simulink model "quadcopter_ctrl_wrench"  (R2024b)
settings: Solver=VariableStepAuto  StartTime=0.0  StopTime=60  RelTol=1e-3
values from neighbouring files (symbols this model uses):
  Ts = 0.001    [params.m]    (also in traj_gen.m)
libraries: robotcorelib x1, uavutilslib x1
settings Model: Creator=feder  LastModifiedBy=mattr

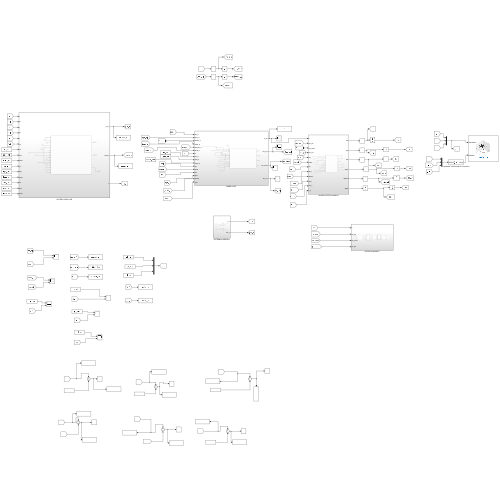
[thumbnail: Simulink's stored preview of the top-level diagram]
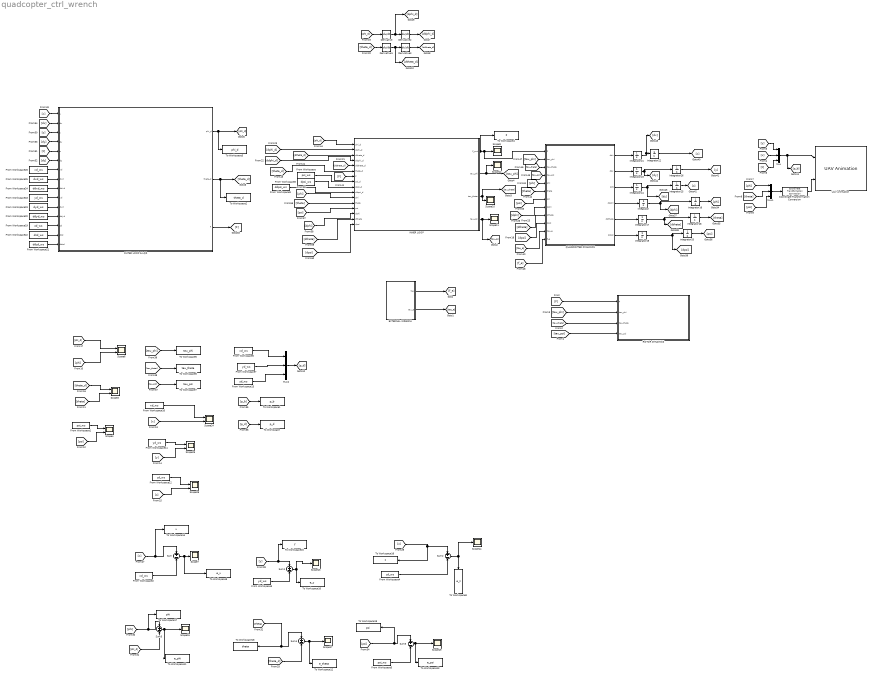
== system quadcopter_ctrl_wrench ==
  Coordinate Transformation Conversion : robotcorelib/Coordinate Transformation Conversion  InputRepresentation=Euler Angles  InputEulerSequence=XYZ  ShowTrVecInputPort=on  OutputRepresentation=Quaternion  OutputEulerSequence=ZYX  ShowTrVecOutputPort=on  SimulateUsing=Interpreted execution
  Derivative : Derivative
  Derivative1 : Derivative  CoefficientInTFapproximation=Ts
  Derivative2 : Derivative
  Derivative3 : Derivative  CoefficientInTFapproximation=Ts
  EXTERNAL WRENCH : Subsystem
  From Workspace : FromWorkspace  VariableName=psi_ws
  From Workspace1 : FromWorkspace  VariableName=psi_ws
  From Workspace{2,6,10,26} (4 alike) : FromWorkspace  VariableName=xd_ws
  From Workspace{3,7,11,18} (4 alike) : FromWorkspace  VariableName=yd_ws
  From Workspace{4,12..13,19} (4 alike) : FromWorkspace  VariableName=zd_ws
  From Workspace20 : FromWorkspace  VariableName=ddyd_ws
  From Workspace21 : FromWorkspace  VariableName=ddzd_ws
  From Workspace22 : FromWorkspace  VariableName=dzd_ws
  From Workspace23 : FromWorkspace  VariableName=dyd_ws
  From Workspace24 : FromWorkspace  VariableName=ddxd_ws
  From Workspace25 : FromWorkspace  VariableName=dxd_ws
  From Workspace5 : FromWorkspace  VariableName=psi_ws
  From Workspace8 : FromWorkspace  VariableName=dpsi_ws
  From Workspace9 : FromWorkspace  VariableName=ddpsi_ws
  INNER LOOP : Subsystem
  Integrator{,17,19,21..26} (9 alike) : Integrator
  Integrator16 : Integrator  InitialCondition=0.09
  Integrator18 : Integrator  InitialCondition=-0.0100316
  Integrator20 : Integrator  InitialCondition=pi/4
  Mux : Mux  Inputs=3
  Mux1 : Mux  Inputs=3
  Mux2 : Mux  Inputs=3
  OUTER LOOP & LQR : Subsystem
  QUADCOPTER DYNAMICS : Subsystem
  ROTOR DYNAMICS : Subsystem
  Scope{7,9..15,17,19} (10 alike) : Scope
  Scope{3..4,6,24..26} (6 alike) : Scope  NumInputPorts=2
  Sum{,1..5} (6 alike) : Sum  Inputs=+-
  To Workspace : ToWorkspace  VariableName=p_d  SaveFormat=Timeseries  SampleTime=-1
  To Workspace1 : ToWorkspace  VariableName=p_b  SaveFormat=Timeseries  SampleTime=-1
  To Workspace10 : ToWorkspace  VariableName=e_y  SaveFormat=Timeseries  SampleTime=-1
  To Workspace11 : ToWorkspace  VariableName=e_phi  SaveFormat=Timeseries  SampleTime=-1
  To Workspace12 : ToWorkspace  VariableName=e_theta  SaveFormat=Timeseries  SampleTime=-1
  To Workspace13 : ToWorkspace  VariableName=e_psi  SaveFormat=Timeseries  SampleTime=-1
  To Workspace14 : ToWorkspace  VariableName=x  SaveFormat=Timeseries  SampleTime=-1
  To Workspace15 : ToWorkspace  VariableName=y  SaveFormat=Timeseries  SampleTime=-1
  To Workspace16 : ToWorkspace  VariableName=z  SaveFormat=Timeseries  SampleTime=-1
  To Workspace17 : ToWorkspace  VariableName=phi  SaveFormat=Timeseries  SampleTime=-1
  To Workspace18 : ToWorkspace  VariableName=theta  SaveFormat=Timeseries  SampleTime=-1
  To Workspace19 : ToWorkspace  VariableName=psi  SaveFormat=Timeseries  SampleTime=-1
  To Workspace2 : ToWorkspace  VariableName=theta_d  SaveFormat=Timeseries  SampleTime=-1
  To Workspace3 : ToWorkspace  VariableName=phi_d  SaveFormat=Timeseries  SampleTime=-1
  To Workspace4 : ToWorkspace  VariableName=F  SaveFormat=Timeseries  SampleTime=-1
  To Workspace5 : ToWorkspace  VariableName=tau_phi  SaveFormat=Timeseries  SampleTime=-1
  To Workspace6 : ToWorkspace  VariableName=tau_theta  SaveFormat=Timeseries  SampleTime=-1
  To Workspace7 : ToWorkspace  VariableName=tau_psi  SaveFormat=Timeseries  SampleTime=-1
  To Workspace8 : ToWorkspace  VariableName=e_z  SaveFormat=Timeseries  SampleTime=-1
  To Workspace9 : ToWorkspace  VariableName=e_x  SaveFormat=Timeseries  SampleTime=-1
  UAV Animation : uavutilslib/UAV Animation  NumUAV=1  DynamicUAVConfig=off  UAVType=Multirotor  UAVSize=1  UAVColor=[1 0 0]  UAVTrajectoryAlpha=1  InertialZDirection=Up  RotationFormat=Quaternion  DrawMarkers=off  SampleTime=0.01
  wires:
  [z] -> Sum2/1, To Workspace16/1
  From Workspace4/1 -> Sum2/2
  Sum2/1 -> Scope14/1, To Workspace8/1
  [x] -> Scope24/2
  From Workspace11/1 -> Scope25/1
  From Workspace10/1 -> Scope24/1
  [phi_d] -> INNER LOOP/1(phi_d)
  [tau_theta] -> QUADCOPTER DYNAMICS/3(tau_theta)
  [theta] -> Scope3/2
  [theta_d] -> Scope3/1
  Mux2/1 -> [p_d]
  [ddtheta_d] -> INNER LOOP/5(ddtheta_d)
  OUTER LOOP & LQR/3(F) -> [F]
  From Workspace21/1 -> OUTER LOOP & LQR/15(ddzd)
  From Workspace19/1 -> OUTER LOOP & LQR/13(zd)
  From Workspace18/1 -> OUTER LOOP & LQR/10(yd)
  [z] -> OUTER LOOP & LQR/5(z)
  From Workspace20/1 -> OUTER LOOP & LQR/12(ddyd)
  [y] -> OUTER LOOP & LQR/3(y)
  [dx] -> OUTER LOOP & LQR/2(dx)
  [x] -> OUTER LOOP & LQR/1(x)
  [tau_psi] -> QUADCOPTER DYNAMICS/4(tau_psi)
  Sum/1 -> To Workspace9/1, Scope7/1
  [z] -> Scope26/2
  [x] -> To Workspace14/1, Sum/1
  [y] -> To Workspace15/1, Sum1/1
  From Workspace3/1 -> Sum1/2
  [phi_d] -> Sum3/2
  Sum1/1 -> Scope13/1, To Workspace10/1
  Sum3/1 -> To Workspace11/1, Scope15/1
  From Workspace2/1 -> Sum/2
  [psi] -> Mux1/3
  QUADCOPTER DYNAMICS/1(ddx) -> Integrator21/1
  QUADCOPTER DYNAMICS/5(ddtheta) -> Integrator17/1
  QUADCOPTER DYNAMICS/4(ddphi) -> Integrator/1
  [dpsi] -> QUADCOPTER DYNAMICS/10(dpsi)
  QUADCOPTER DYNAMICS/3(ddz) -> Integrator24/1
  [y] -> Scope25/2
  QUADCOPTER DYNAMICS/6(ddpsi) -> Integrator19/1
  QUADCOPTER DYNAMICS/2(ddy) -> Integrator23/1
  [theta] -> QUADCOPTER DYNAMICS/6(theta)
  [phi] -> QUADCOPTER DYNAMICS/5(phi)
  [dtheta] -> QUADCOPTER DYNAMICS/9(dtheta)
  [dphi] -> QUADCOPTER DYNAMICS/8(dphi)
  [psi] -> QUADCOPTER DYNAMICS/7(psi)
  [dpsi] -> INNER LOOP/16(dpsi)
  INNER LOOP/3(tau_theta) -> Scope10/1, [tau_theta]
  INNER LOOP/2(tau_phi) -> [tau_phi], Scope12/1
  INNER LOOP/4(tau_psi) -> Scope11/1, [tau_psi]
  INNER LOOP/1(F_out) -> To Workspace4/1, QUADCOPTER DYNAMICS/1(F), Scope9/1
  [theta] -> INNER LOOP/12(theta)
  [psi] -> INNER LOOP/13(psi)
  [dtheta] -> INNER LOOP/15(dtheta)
  [phi] -> INNER LOOP/11(phi)
  From Workspace9/1 -> INNER LOOP/10(ddpsi_d)
  From Workspace8/1 -> INNER LOOP/9(dpsi_d)
  From Workspace/1 -> INNER LOOP/8(psi_d)
  [F] -> INNER LOOP/7(F)
  [ddphi_d] -> INNER LOOP/4(ddphi_d)
  [dtheta_d] -> INNER LOOP/3(dtheta_d)
  [tau_phi] -> QUADCOPTER DYNAMICS/2(tau_phi)
  [dz] -> OUTER LOOP & LQR/6(dz)
  From Workspace1/1 -> Scope4/1
  [theta_d] -> Derivative1/1
  [phi] -> Scope6/2
  [y] -> Mux/1
  [phi] -> Mux1/1
  Integrator20/1 -> [psi]
  Derivative/1 -> [dphi_d], Derivative2/1
  Integrator25/1 -> [z]
  Mux1/1 -> Coordinate Transformation Conversion/1
  Integrator19/1 -> [dpsi], Integrator20/1
  From Workspace24/1 -> OUTER LOOP & LQR/9(ddxd)
  [dphi_d] -> INNER LOOP/2(dphi_d)
  Integrator26/1 -> [y]
  Integrator/1 -> [dphi], Integrator16/1
  [phi_d] -> Derivative/1
  Integrator17/1 -> [dtheta], Integrator18/1
  [theta] -> Mux1/2
  Integrator18/1 -> [theta]
  From Workspace22/1 -> OUTER LOOP & LQR/14(dzd)
  From Workspace25/1 -> OUTER LOOP & LQR/8(dxd)
  Integrator21/1 -> [dx], Integrator22/1
  From Workspace23/1 -> OUTER LOOP & LQR/11(dyd)
  Integrator16/1 -> [phi]
  Derivative2/1 -> [ddphi_d]
  Coordinate Transformation Conversion/1 -> UAV Animation/2
  Derivative3/1 -> [ddtheta_d]
  [dy] -> OUTER LOOP & LQR/4(dy)
  [phi] -> To Workspace17/1, Sum3/1
  From Workspace12/1 -> Scope26/1
  [tau_phi] -> To Workspace5/1
  Derivative1/1 -> [dtheta_d], Derivative3/1
  Integrator22/1 -> [x]
  [z] -> Mux/3
  [x] -> Mux/2
  Integrator23/1 -> [dy], Integrator26/1
  [theta] -> To Workspace18/1, Sum4/1
  [theta_d] -> Sum4/2
  Mux/1 -> [p_b], UAV Animation/1
  From Workspace5/1 -> Sum5/2
  Integrator24/1 -> [dz], Integrator25/1
  [dphi] -> INNER LOOP/14(dphi)
  Sum4/1 -> To Workspace12/1, Scope17/1
  [psi] -> Sum5/1, To Workspace19/1
  From Workspace7/1 -> Mux2/2
  [p_d] -> To Workspace/1
  OUTER LOOP & LQR/2(theta_d) -> To Workspace2/1, [theta_d]
  [tau_theta] -> To Workspace6/1
  From Workspace26/1 -> OUTER LOOP & LQR/7(xd)
  [p_b] -> To Workspace1/1
  From Workspace13/1 -> Mux2/3
  [F] -> ROTOR DYNAMICS/1(F)
  [tau_theta] -> ROTOR DYNAMICS/3(tau_theta)
  [tau_psi] -> ROTOR DYNAMICS/4(tau_psi)
  [phi_d] -> Scope6/1
  Sum5/1 -> To Workspace13/1, Scope19/1
  [tau_phi] -> ROTOR DYNAMICS/2(tau_phi)
  [tau_psi] -> To Workspace7/1
  OUTER LOOP & LQR/1(phi_d) -> [phi_d], To Workspace3/1
  [psi] -> Scope4/2
  From Workspace6/1 -> Mux2/1
  [theta_d] -> INNER LOOP/6(theta_d)
  [tau_e] -> QUADCOPTER DYNAMICS/11(tau_e)
  [f_e] -> QUADCOPTER DYNAMICS/12(f_e)
  EXTERNAL WRENCH/1(f_e) -> [f_e]
  EXTERNAL WRENCH/2(tau_e) -> [tau_e]

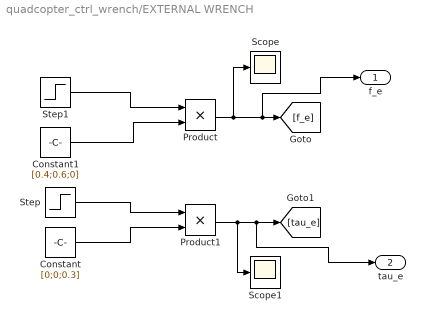
== system quadcopter_ctrl_wrench/EXTERNAL WRENCH ==
  Constant : Constant  Value=[0;0;0.3]  SampleTime=Ts
  Constant1 : Constant  Value=[0.4;0.6;0]  SampleTime=Ts
  Product : Product
  Product1 : Product
  Scope : Scope
  Scope1 : Scope
  Step : Step  Time=12  SampleTime=Ts
  Step1 : Step  Time=12  SampleTime=Ts
  f_e : Outport
  tau_e : Outport  Port=2
  wires:
  Product/1 -> Scope/1, f_e/1, [f_e]
  Product1/1 -> Scope1/1, tau_e/1, [tau_e]
  Step1/1 -> Product/1
  Constant1/1 -> Product/2
  Step/1 -> Product1/1
  Constant/1 -> Product1/2

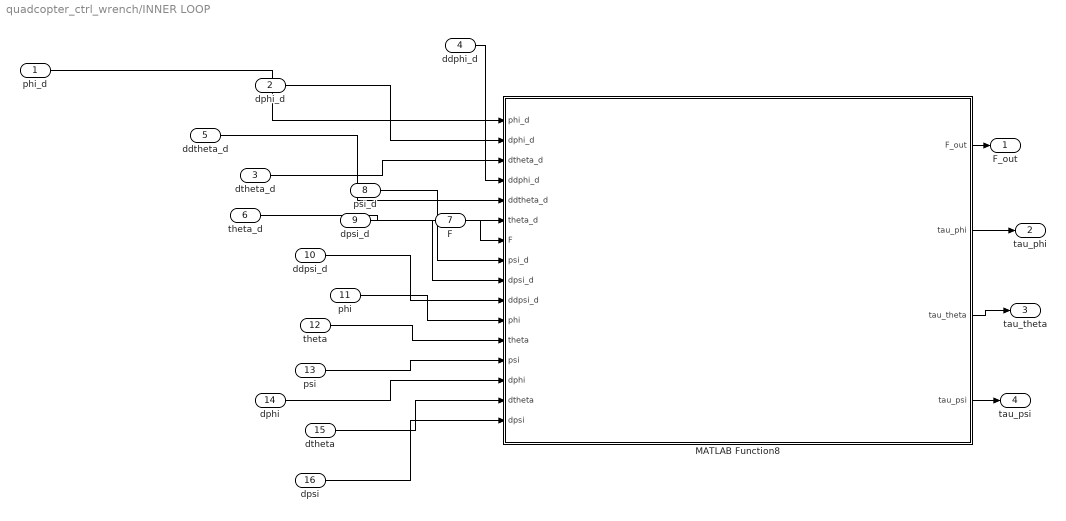
== system quadcopter_ctrl_wrench/INNER LOOP ==
  phi_d : Inport
  dphi_d : Inport  Port=2
  dtheta_d : Inport  Port=3
  ddphi_d : Inport  Port=4
  ddtheta_d : Inport  Port=5
  theta_d : Inport  Port=6
  F : Inport  Port=7
  psi_d : Inport  Port=8
  dpsi_d : Inport  Port=9
  ddpsi_d : Inport  Port=10
  phi : Inport  Port=11
  theta : Inport  Port=12
  psi : Inport  Port=13
  dphi : Inport  Port=14
  dtheta : Inport  Port=15
  dpsi : Inport  Port=16
  MATLAB Function8 : MATLAB Function  TreatAsAtomicUnit=on
  F_out : Outport
  tau_phi : Outport  Port=2
  tau_theta : Outport  Port=3
  tau_psi : Outport  Port=4
  wires:
  ddphi_d/1 -> MATLAB Function8/4(ddphi_d)
  psi_d/1 -> MATLAB Function8/8(psi_d)
  ddpsi_d/1 -> MATLAB Function8/10(ddpsi_d)
  F/1 -> MATLAB Function8/7(F)
  psi/1 -> MATLAB Function8/13(psi)
  dphi_d/1 -> MATLAB Function8/2(dphi_d)
  dphi/1 -> MATLAB Function8/14(dphi)
  phi_d/1 -> MATLAB Function8/1(phi_d)
  MATLAB Function8/1(F_out) -> F_out/1
  phi/1 -> MATLAB Function8/11(phi)
  dpsi_d/1 -> MATLAB Function8/9(dpsi_d)
  ddtheta_d/1 -> MATLAB Function8/5(ddtheta_d)
  theta/1 -> MATLAB Function8/12(theta)
  MATLAB Function8/2(tau_phi) -> tau_phi/1
  MATLAB Function8/3(tau_theta) -> tau_theta/1
  dtheta_d/1 -> MATLAB Function8/3(dtheta_d)
  dtheta/1 -> MATLAB Function8/15(dtheta)
  MATLAB Function8/4(tau_psi) -> tau_psi/1
  theta_d/1 -> MATLAB Function8/6(theta_d)
  dpsi/1 -> MATLAB Function8/16(dpsi)

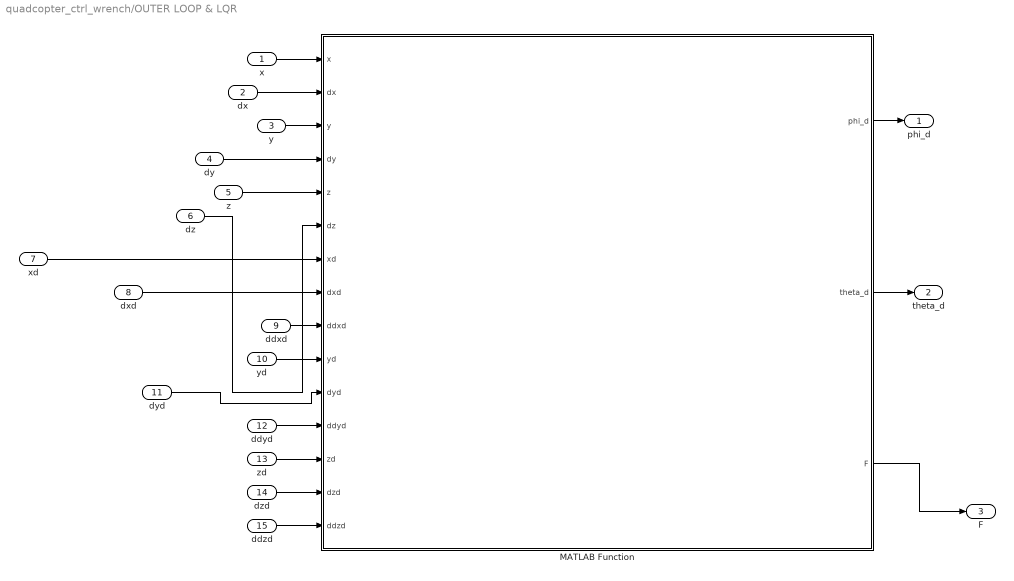
== system quadcopter_ctrl_wrench/OUTER LOOP & LQR ==
  x : Inport
  dx : Inport  Port=2
  y : Inport  Port=3
  dy : Inport  Port=4
  z : Inport  Port=5
  dz : Inport  Port=6
  xd : Inport  Port=7
  dxd : Inport  Port=8
  ddxd : Inport  Port=9
  yd : Inport  Port=10
  dyd : Inport  Port=11
  ddyd : Inport  Port=12
  zd : Inport  Port=13
  dzd : Inport  Port=14
  ddzd : Inport  Port=15
  MATLAB Function : MATLAB Function  TreatAsAtomicUnit=on
  phi_d : Outport
  theta_d : Outport  Port=2
  F : Outport  Port=3
  wires:
  zd/1 -> MATLAB Function/13(zd)
  MATLAB Function/1(phi_d) -> phi_d/1
  xd/1 -> MATLAB Function/7(xd)
  dxd/1 -> MATLAB Function/8(dxd)
  dy/1 -> MATLAB Function/4(dy)
  MATLAB Function/2(theta_d) -> theta_d/1
  dyd/1 -> MATLAB Function/11(dyd)
  ddzd/1 -> MATLAB Function/15(ddzd)
  dz/1 -> MATLAB Function/6(dz)
  yd/1 -> MATLAB Function/10(yd)
  dx/1 -> MATLAB Function/2(dx)
  dzd/1 -> MATLAB Function/14(dzd)
  y/1 -> MATLAB Function/3(y)
  ddxd/1 -> MATLAB Function/9(ddxd)
  z/1 -> MATLAB Function/5(z)
  ddyd/1 -> MATLAB Function/12(ddyd)
  x/1 -> MATLAB Function/1(x)
  MATLAB Function/3(F) -> F/1

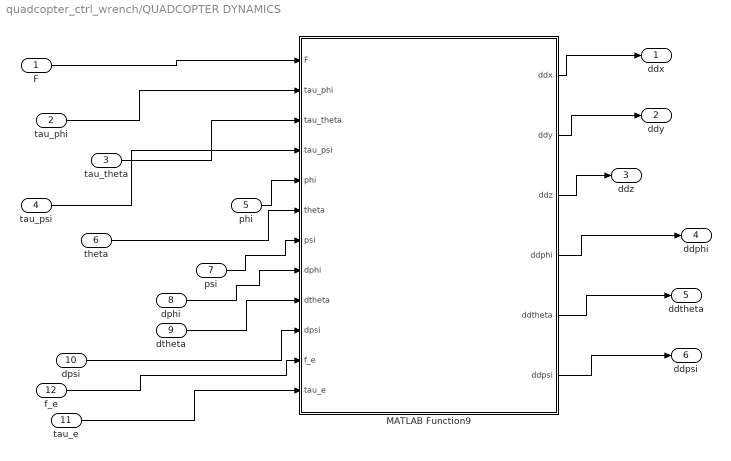
== system quadcopter_ctrl_wrench/QUADCOPTER DYNAMICS ==
  F : Inport
  tau_phi : Inport  Port=2
  tau_theta : Inport  Port=3
  tau_psi : Inport  Port=4
  phi : Inport  Port=5
  theta : Inport  Port=6
  psi : Inport  Port=7
  dphi : Inport  Port=8
  dtheta : Inport  Port=9
  dpsi : Inport  Port=10
  tau_e : Inport  Port=11
  f_e : Inport  Port=12
  MATLAB Function9 : MATLAB Function  TreatAsAtomicUnit=on
  ddx : Outport
  ddy : Outport  Port=2
  ddz : Outport  Port=3
  ddphi : Outport  Port=4
  ddtheta : Outport  Port=5
  ddpsi : Outport  Port=6
  wires:
  dphi/1 -> MATLAB Function9/8(dphi)
  MATLAB Function9/6(ddpsi) -> ddpsi/1
  phi/1 -> MATLAB Function9/5(phi)
  MATLAB Function9/2(ddy) -> ddy/1
  tau_phi/1 -> MATLAB Function9/2(tau_phi)
  MATLAB Function9/4(ddphi) -> ddphi/1
  F/1 -> MATLAB Function9/1(F)
  dtheta/1 -> MATLAB Function9/9(dtheta)
  MATLAB Function9/3(ddz) -> ddz/1
  tau_theta/1 -> MATLAB Function9/3(tau_theta)
  MATLAB Function9/1(ddx) -> ddx/1
  MATLAB Function9/5(ddtheta) -> ddtheta/1
  theta/1 -> MATLAB Function9/6(theta)
  dpsi/1 -> MATLAB Function9/10(dpsi)
  tau_psi/1 -> MATLAB Function9/4(tau_psi)
  psi/1 -> MATLAB Function9/7(psi)
  tau_e/1 -> MATLAB Function9/12(tau_e)
  f_e/1 -> MATLAB Function9/11(f_e)

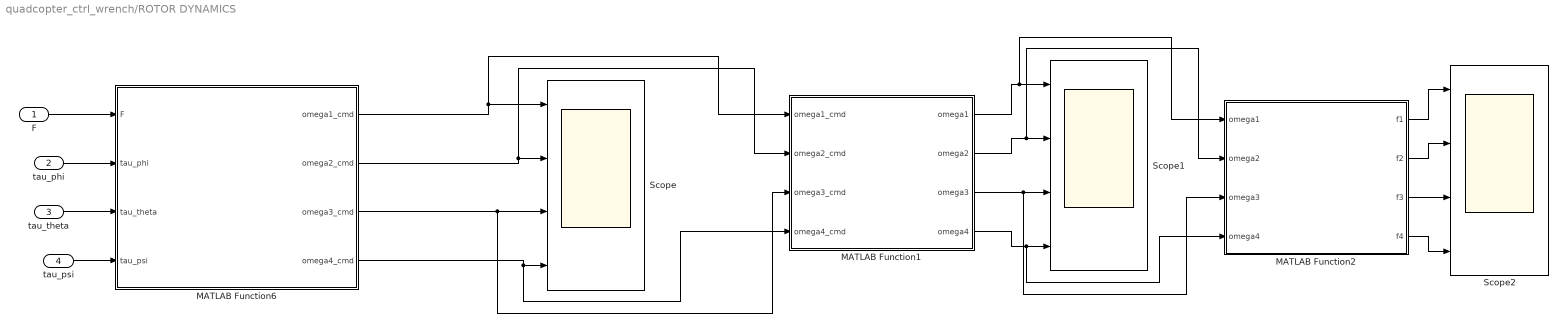
== system quadcopter_ctrl_wrench/ROTOR DYNAMICS ==
  F : Inport
  tau_phi : Inport  Port=2
  tau_theta : Inport  Port=3
  tau_psi : Inport  Port=4
  MATLAB Function1 : MATLAB Function  TreatAsAtomicUnit=on
  MATLAB Function2 : MATLAB Function  TreatAsAtomicUnit=on
  MATLAB Function6 : MATLAB Function  TreatAsAtomicUnit=on
  Scope : Scope  NumInputPorts=4
  Scope1 : Scope  NumInputPorts=4
  Scope2 : Scope  NumInputPorts=4
  wires:
  MATLAB Function6/3(omega3_cmd) -> MATLAB Function1/3(omega3_cmd), Scope/3
  MATLAB Function1/1(omega1) -> MATLAB Function2/1(omega1), Scope1/1
  MATLAB Function2/3(f3) -> Scope2/3
  F/1 -> MATLAB Function6/1(F)
  MATLAB Function1/4(omega4) -> MATLAB Function2/4(omega4), Scope1/4
  MATLAB Function2/4(f4) -> Scope2/4
  MATLAB Function6/4(omega4_cmd) -> MATLAB Function1/4(omega4_cmd), Scope/4
  MATLAB Function2/1(f1) -> Scope2/1
  MATLAB Function1/3(omega3) -> MATLAB Function2/3(omega3), Scope1/3
  MATLAB Function2/2(f2) -> Scope2/2
  MATLAB Function6/1(omega1_cmd) -> MATLAB Function1/1(omega1_cmd), Scope/1
  MATLAB Function1/2(omega2) -> MATLAB Function2/2(omega2), Scope1/2
  MATLAB Function6/2(omega2_cmd) -> MATLAB Function1/2(omega2_cmd), Scope/2
  tau_psi/1 -> MATLAB Function6/4(tau_psi)
  tau_theta/1 -> MATLAB Function6/3(tau_theta)
  tau_phi/1 -> MATLAB Function6/2(tau_phi)

== matlab function quadcopter_ctrl_wrench/QUADCOPTER DYNAMICS/MATLAB Function9 ==
  settings: updateMethod=DISCRETE
  data: F input; ddx output; ddy output; ddz output; tau_phi input; ddphi output; tau_theta input; tau_psi input; phi input; theta input; psi input; ddtheta output; ddpsi output; dphi input; dtheta input; dpsi input; f_e input; tau_e input
function [ddx, ddy, ddz, ddphi, ddtheta, ddpsi] = QuadcopterDynamics(F, tau_phi, tau_theta, tau_psi, ...
 phi, theta, psi, dphi, dtheta, dpsi, f_e, tau_e)


persistent m g J params_loaded
if isempty(params_loaded)
    params = load('quadcopter_params.mat', 'm', 'g', 'J');
    m = params.m;
    g = params.g;
    J = params.J;
    params_loaded = true;
end

c_phi = cos(phi); s_phi = sin(phi);
c_theta = cos(theta); s_theta = sin(theta);
c_psi = cos(psi); s_psi = sin(psi);

R_eb = [c_psi*c_theta, -c_theta*s_psi, s_theta;
        c_phi*s_psi + c_psi*s_phi*s_theta, c_phi*c_psi - s_phi*s_psi*s_theta, -c_theta*s_phi;
        s_phi*s_psi - c_phi*c_psi*s_theta, c_psi*s_phi + c_phi*s_psi*s_theta, c_phi*c_theta];

F_body = [0; 0; F];
F_inertial = R_eb * F_body + [0; 0; -m*g] + (1/m)*f_e;
dd_pos = F_inertial / m;

ddx = dd_pos(1);
ddy = dd_pos(2);
ddz = dd_pos(3);

W_n = [1, 0, -s_theta;
       0, c_phi, c_theta*s_phi;
       0, -s_phi, c_theta*c_phi];

if abs(cos(theta)) < 1e-6
    warning('Singolarità in W_n, uso approssimazione');
    dd_angles = J \ [tau_phi; tau_theta; tau_psi];
else
    J_tilde = J * W_n;
    
    Ixx = J(1,1);
    Iyy = J(2,2);
    Izz = J(3,3);
    
    omega_body = W_n * [dphi; dtheta; dpsi];
    p = omega_body(1);
    q = omega_body(2);  
    r = omega_body(3);
    
    C_term = [q*r*(Izz - Iyy);
              p*r*(Ixx - Izz);
              p*q*(Iyy - Ixx)];

    tau_vec = [tau_phi; tau_theta; tau_psi];
    dd_angles = J_tilde \ (tau_vec - C_term + tau_e);
end

ddphi = dd_angles(1);
ddtheta = dd_angles(2);
ddpsi = dd_angles(3);


max_lin_acc = 0.5; 
max_ang_acc = 1; 

ddx = max(-max_lin_acc, min(ddx, max_lin_acc));
ddy = max(-max_lin_acc, min(ddy, max_lin_acc));
ddz = max(-max_lin_acc, min(ddz, max_lin_acc));
ddphi = max(-max_ang_acc, min(ddphi, max_ang_acc));
ddtheta = max(-max_ang_acc, min(ddtheta, max_ang_acc));
ddpsi = max(-max_ang_acc, min(ddpsi, max_ang_acc));
end

== matlab function quadcopter_ctrl_wrench/ROTOR DYNAMICS/MATLAB Function1 ==
  data: omega1_cmd input; omega1 output; omega2_cmd input; omega3_cmd input; omega4_cmd input; omega2 output; omega3 output; omega4 output
function [omega1, omega2, omega3, omega4] = ESC_Model(omega1_cmd, omega2_cmd, omega3_cmd, omega4_cmd)

persistent omega_prev params_loaded tau_esc omega_max dt

if isempty(params_loaded)
    tau_esc = 0.03;
    omega_max = 1200;
    dt = 0.001;
    
    omega_prev = [0; 0; 0; 0];
    
    params_loaded = true;
end

omega_cmd = [omega1_cmd; omega2_cmd; omega3_cmd; omega4_cmd];

omega_cmd = max(0, min(omega_cmd, omega_max));

alpha = dt / (tau_esc + dt);
omega_new = alpha * omega_cmd + (1-alpha) * omega_prev;

omega_new = max(0, min(omega_new, omega_max));

omega1 = omega_new(1);
omega2 = omega_new(2);
omega3 = omega_new(3);
omega4 = omega_new(4);

omega_prev = omega_new;
end

== matlab function quadcopter_ctrl_wrench/OUTER LOOP & LQR/MATLAB Function ==
  data: x input; phi_d output; dx input; y input; dy input; z input; dz input; xd input; dxd input; ddxd input; yd input; dyd input; ddyd input; zd input; dzd input; ddzd input; theta_d output; F output
function [phi_d, theta_d, F] = OuterLQR(x, dx, y, dy, z, dz, ...
                                       xd, dxd, ddxd, ...
                                       yd, dyd, ddyd, ...
                                       zd, dzd, ddzd)
persistent K_loaded K m g

if isempty(K_loaded)
    S = load('quadcopter_params.mat', 'K', 'm', 'g'); 
    K = S.K;
    m = S.m;
    g = S.g;
    K_loaded = true;
end

xi = [x; dx; y; dy; z; dz];
xi_d = [xd; dxd; yd; dyd; zd; dzd];

e = xi - xi_d;
r_hat = -K * e;

r = [ddxd; ddyd; ddzd] + r_hat;


rx = r(1); ry = r(2); rz = r(3);


phi_d = atan(-ry / (rz + g));
theta_d = atan(rx * cos(phi_d) / (rz + g)); 
F = m * (rz + g) / (cos(theta_d) * cos(phi_d));
end

== matlab function quadcopter_ctrl_wrench/ROTOR DYNAMICS/MATLAB Function2 ==
  data: omega1 input; f1 output; omega2 input; omega3 input; omega4 input; f2 output; f3 output; f4 output
function [f1, f2, f3, f4] = RotorPropellerDynamics(omega1, omega2, omega3, omega4)
persistent k params_loaded

if isempty(params_loaded)
    params = load('quadcopter_params.mat', 'k');
    k = params.k;
    params_loaded = true;
end

f1 = k * omega1^2;
f2 = k * omega2^2;
f3 = k * omega3^2;
f4 = k * omega4^2;
end

== matlab function quadcopter_ctrl_wrench/ROTOR DYNAMICS/MATLAB Function6 ==
  settings: updateMethod=DISCRETE
  data: F input; omega1_cmd output; tau_phi input; tau_theta input; tau_psi input; omega2_cmd output; omega3_cmd output; omega4_cmd output
function [omega1_cmd, omega2_cmd, omega3_cmd, omega4_cmd] = AngularVelocityConversion(F, tau_phi, tau_theta, tau_psi)

persistent L k b m g mixing_inv params_loaded

if isempty(params_loaded)
    params = load('quadcopter_params.mat', 'm', 'g', 'L', 'k', 'b');
    m = params.m;
    g = params.g;
    L = params.L;
    k = params.k;
    b = params.b;
  
    
    L_sqrt2 = L / sqrt(2);
    
    mixing = [1, 1, 1, 1;
              L_sqrt2, -L_sqrt2, -L_sqrt2, L_sqrt2;
              -L_sqrt2, -L_sqrt2, L_sqrt2, L_sqrt2;
              -b/k, b/k, -b/k, b/k];
    
    if abs(det(mixing)) < 1e-10
        error('Mixing matrix è singolare! Verifica configurazione motori.');
    end
    
    mixing_inv = inv(mixing);
    params_loaded = true;
end

F_max = 4 * m * g;
tau_max = 2;

F = max(0.1, min(F, F_max));
tau_phi = max(-tau_max, min(tau_phi, tau_max));
tau_theta = max(-tau_max, min(tau_theta, tau_max));
tau_psi = max(-tau_max, min(tau_psi, tau_max));

commands = [F; tau_phi; tau_theta; tau_psi];
forces = mixing_inv * commands;

f1 = max(0.01, forces(1));
f2 = max(0.01, forces(2));
f3 = max(0.01, forces(3));
f4 = max(0.01, forces(4));

omega1_cmd = sqrt(f1 / k);
omega2_cmd = sqrt(f2 / k);
omega3_cmd = sqrt(f3 / k);
omega4_cmd = sqrt(f4 / k);

omega_max = 1000;
omega1_cmd = min(omega1_cmd, omega_max);
omega2_cmd = min(omega2_cmd, omega_max);
omega3_cmd = min(omega3_cmd, omega_max);
omega4_cmd = min(omega4_cmd, omega_max);
end

== matlab function quadcopter_ctrl_wrench/INNER LOOP/MATLAB Function8 ==
  data: phi_d input; dphi_d input; dtheta_d input; ddphi_d input; ddtheta_d input; theta_d input; F input; psi_d input; dpsi_d input; ddpsi_d input; F_out output; phi input; tau_phi output; theta input; psi input; dphi input; dtheta input; dpsi input; tau_theta output; tau_psi output
function [F_out, tau_phi, tau_theta, tau_psi] = InnerLoop(phi_d,dphi_d,dtheta_d,ddphi_d, ddtheta_d,theta_d, F, ...
 psi_d, dpsi_d, ddpsi_d, ...
 phi, theta, psi, ...
 dphi, dtheta, dpsi)


persistent k1_phi k2_phi k1_theta k2_theta k1_psi k2_psi J_mat gains_loaded
if isempty(gains_loaded)
    params_struct = load('quadcopter_params.mat', 'k1_phi', 'k2_phi', 'k1_theta', 'k2_theta', 'k1_psi', 'k2_psi', 'J');
    k1_phi = params_struct.k1_phi;
    k2_phi = params_struct.k2_phi;
    k1_theta = params_struct.k1_theta;
    k2_theta = params_struct.k2_theta;
    k1_psi = params_struct.k1_psi;
    k2_psi = params_struct.k2_psi;
    J_mat = params_struct.J;
    gains_loaded = true;
end

e_phi = phi - phi_d;
de_phi = dphi - dphi_d;
e_theta = theta - theta_d;
de_theta = dtheta - dtheta_d;
e_psi = psi - psi_d;
de_psi = dpsi - dpsi_d;

tau_tilde_phi = ddphi_d - k2_phi * de_phi - k1_phi * e_phi;
tau_tilde_theta = ddtheta_d - k2_theta * de_theta - k1_theta * e_theta;
tau_tilde_psi = ddpsi_d - k2_psi * de_psi - k1_psi * e_psi;

c_phi = cos(phi); s_phi = sin(phi);
c_theta = cos(theta); s_theta = sin(theta);

W_n = [1, 0, -s_theta;
       0, c_phi, c_theta*s_phi;
       0, -s_phi, c_theta*c_phi];

if abs(cos(theta)) < 1e-6
    warning('Singolarità in W_n durante controllo');
    tau_physical = J_mat * [tau_tilde_phi; tau_tilde_theta; tau_tilde_psi];
else
    J_tilde = J_mat * W_n;

    tau_tilde_vec = [tau_tilde_phi; tau_tilde_theta; tau_tilde_psi];
    tau_physical = J_tilde * tau_tilde_vec;
end

tau_phi = tau_physical(1);
tau_theta = tau_physical(2);
tau_psi = tau_physical(3);

F_out = F;

tau_max_phi=8;
tau_max_theta = 10;
tau_max_psi=8;
tau_phi = max(-tau_max_phi, min(tau_phi, tau_max_phi));
tau_theta = max(-tau_max_theta, min(tau_theta, tau_max_theta));
tau_psi = max(-tau_max_psi, min(tau_psi, tau_max_psi));

end
